simulink model "asbCubeSat"  (R2025b)
settings: Solver=VariableStepAuto  StartTime=0.0  StopTime=10800  FixedStep=CubeSatTimeStep  MaxStep=10  RelTol=1e-7  AbsTol=1e-7  EnableMultiTasking=on
libraries: simulink x12, aerolibutil x5, asbCubeSatEnvironmentLib x1, SignalEditorBlockLib x1, sharedutil x1, asbCubeSatActuatorsLib x1, asbCubeSatSensorsLib x1, asbCubeSatDynamicsLib x1, asbCubeSatFSWLib x1
settings Model: RequirementInfo={} %GIDa_aedc6be2_fb6a_446c_8c25_10b8bc9db182  DataDictionary=asbCubeSatModelData.sldd  SnapshotInterval=1  ExtModeAutoUpdateStatusClock=off  Creator=The MathWorks, Inc.  LastModifiedBy=The MathWorks, Inc.
settings SolverCC: AlgebraicLoopSolver=TrustRegion  MaxZcPerStep=1.0
settings DataIOCC: LimitDataPoints=on  SaveFormat=Array  SaveOutput=off  DSMLogging=off  SaveTime=off  ReturnWorkspaceOutputs=off
settings OptimizationCC: DefaultParameterBehavior=Inlined  OptimizeBlockIOStorage=off  BufferReuse=off  GlobalBufferReuse=off  ExpressionFolding=off  ExpressionDepthLimit=2147483647.0  LocalBlockOutputs=off  InitFltsAndDblsToZero=on  LifeSpan=inf  OptimizeDataStoreBuffers=off  BusAssignmentInplaceUpdate=off
settings DebuggingCC: SignalResolutionControl=TryResolveAllWithWarning  MultiTaskDSMMsg=warning  MultiTaskCondExecSysMsg=none  UnconnectedInputMsg=warning  UnconnectedOutputMsg=warning  UnconnectedLineMsg=warning  AssertControl=DisableAll  StateNameClashWarn=warning  PregeneratedLibrarySubsystemCodeDiagnostic=none  SFUnexpectedBacktrackingDiag=warning  SFNoUnconditionalDefaultTransitionDiag=warning  SFExecutionAtInitializationDiag=none  ArithmeticOperatorsInVariantConditions=warning
settings HardwareCC: ProdBitPerPointer=32.0  ProdBitPerSizeT=32.0  ProdBitPerPtrDiffT=32.0  ProdLargestAtomicFloat=None  ProdIntDivRoundTo=Undefined  ProdEndianess=Unspecified  ProdWordSize=32.0  ProdHWDeviceType=32-bit Generic
settings ModelReferenceCC: UpdateModelReferenceTargets=IfOutOfDate  EnableRefExpFcnMdlSchedulingChecks=on  ModelReferenceMinAlgLoopOccurrences=on  PropagateSignalLabelsOutOfModel=off
settings SFSimCC: SimUseLocalCustomCode=off
settings RTWCC: RTWUseLocalCustomCode=off  GPUComputeCapability=3.5  DLArmComputeVersion=19.05
settings CodeAppCC: StateflowObjectComments=on
settings GRTTargetCC: TargetFcnLib=ansi_tfl_tmw.mat  TargetLangStandard=C89/C90 (ANSI)  CombineOutputUpdateFcns=off  GRTInterface=on
settings ConfigComp: CovMetricSettings=dw  CovSaveCumulativeToWorkspaceVar=on  CovSaveSingleToWorkspaceVar=on  CovExternalEMLEnable=off

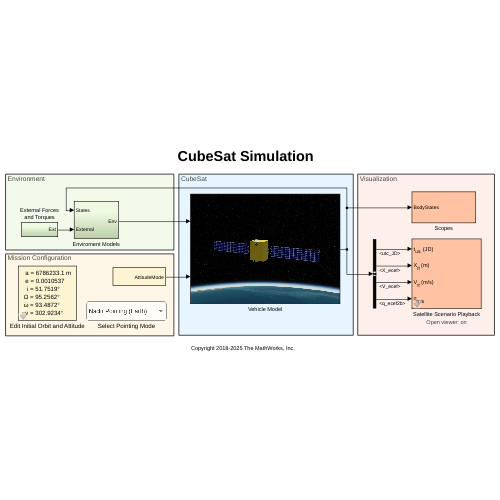
[thumbnail: Simulink's stored preview of the top-level diagram]
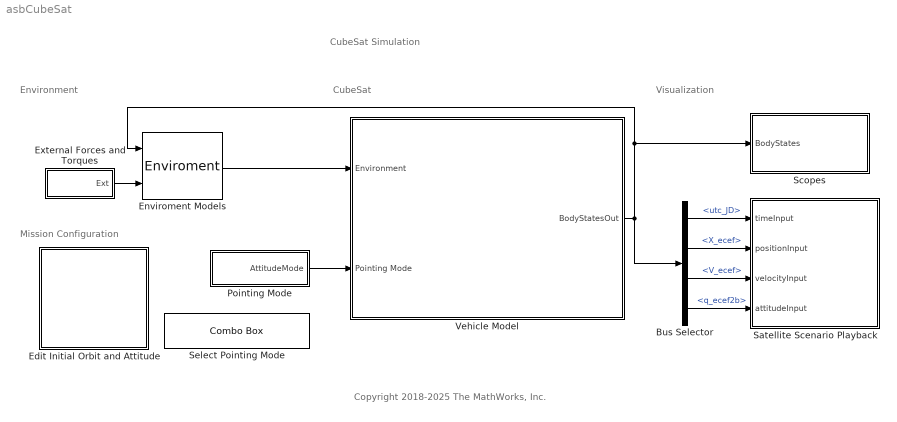
== system asbCubeSat ==
  note: Visualization
  note: CubeSat
  note: Environment
  note: Copyright 2018-2025 The MathWorks, Inc.
  note: CubeSat Simulation
  note: Mission Configuration
  Bus Selector : BusSelector  OutputSignals=utc_JD,X_ecef,V_ecef,q_ecef2b
  Edit Initial Orbit and Attitude : Subsystem  mask(CubeSat Initial Conditions){sim_t0=2458488, epoch=2451545, method=Keplerian Orbital Elements, a=6786233.13, ecc=0.0010537, incl=51.7519, omega=95.2562, argp=93.4872, nu=302.9234, truelon=0, arglat=0, lonper=0, r_eci=[-2981784.257 5207055.9381 3161595.3068], v_eci=[-3384.4834 -4887.7595 4843.4609], r_ecef=[-5762650.9114 -1682704.282 3156028.2879], v_ecef=[3832.57 -4024.9014 4837.4311], lla=[27.88080034 -163.722102 408851.6223], v_ned=[5468.7396 4937.8129 -7.4627367], euler=[33.9 -5.91 9.88], pqr=[0 0 0]}
      mask prompts: sim_t0 "spacecraft:cubesat:StartDate"; epoch "spacecraft:cubesat:ECIEpoch"; method "spacecraft:cubesat:InputMethod"; a "spacecraft:cubesat:SemiMajorAxis"; ecc "spacecraft:cubesat:Eccentricity"; incl "spacecraft:cubesat:Inclination"; omega "spacecraft:cubesat:RAAN"; argp "spacecraft:cubesat:ArgP"; nu "spacecraft:cubesat:TrueAnomaly"; truelon "spacecraft:cubesat:TrueLon"; arglat "spacecraft:cubesat:ArgLat"; lonper "spacecraft:cubesat:LonPer"; r_eci "spacecraft:cubesat:ECIPos"; v_eci "spacecraft:cubesat:ECIVel"; r_ecef "spacecraft:cubesat:ECEFPos"; v_ecef "spacecraft:cubesat:ECEFVel"; lla "spacecraft:cubesat:LLA"; v_ned "spacecraft:cubesat:NEDVel"; euler "spacecraft:cubesat:Euler"; pqr "spacecraft:cubesat:BodyAngRates"
      mask help: spacecraft:cubesat:InitCondBlockDesc
      mask init:
      | initCond = cubeSatCallback(gcb, 'computeIC', method, sim_t0, epoch, a, ecc, incl,...
      |     omega, argp, nu, truelon, arglat, lonper, r_eci, v_eci, r_ecef, v_ecef, lla,...
      |     v_ned, euler, pqr);
      mask TypeOptions method: spacecraft:cubesat:InputKeplerian | spacecraft:cubesat:InputECI | spacecraft:cubesat:InputECEF | spacecraft:cubesat:InputLLANED
      mask Callback method: cubeSatCallback(gcb, 'handleMethod');
      mask Callback ecc: cubeSatCallback(gcb, 'handleCircularOrbit');
      mask Callback incl: cubeSatCallback(gcb, 'handleCircularOrbit');
      mask DialogControl sim_t0 Prompt: Start date [Julian date]:
      mask DialogControl sim_t0 Tooltip: spacecraft:spacecraft:StartDateTT
      mask DialogControl icTab Prompt: spacecraft:cubesat:InitCond
      mask DialogControl epoch Prompt: Epoch of ECI frame [Julian date]:
      mask DialogControl epoch Tooltip: spacecraft:cubesat:ECIEpochTT
      mask DialogControl Container9 Prompt: spacecraft:cubesat:InitCondOrbit
      mask DialogControl method Prompt: Input method:
      mask DialogControl method Tooltip: spacecraft:cubesat:InputMethodTT
      mask DialogControl a Prompt: Semi-major axis [m]:
      mask DialogControl a Tooltip: spacecraft:cubesat:SemiMajorAxisTT
      mask DialogControl ecc Prompt: Eccentricity:
      mask DialogControl ecc Tooltip: spacecraft:cubesat:EccentricityTT
      mask DialogControl incl Prompt: Inclination [deg]:
      mask DialogControl incl Tooltip: spacecraft:cubesat:InclinationTT
      mask DialogControl omega Prompt: Right ascension of the ascending node [deg]:
      mask DialogControl omega Tooltip: spacecraft:cubesat:RAANTT
      mask DialogControl argp Prompt: Argument of periapsis [deg]:
      mask DialogControl argp Tooltip: spacecraft:cubesat:ArgPTT
      mask DialogControl nu Prompt: True anomaly [deg]:
      mask DialogControl nu Tooltip: spacecraft:cubesat:TrueAnomalyTT
      mask DialogControl truelon Prompt: True longitude [deg] (circular equatorial):
      mask DialogControl truelon Tooltip: spacecraft:cubesat:TrueLonTT
      mask DialogControl arglat Prompt: Argument of latitude [deg] (circular inclined):
      mask DialogControl arglat Tooltip: spacecraft:cubesat:ArgLatTT
      mask DialogControl lonper Prompt: Longitude of periapsis [deg] (elliptical equatorial):
      mask DialogControl lonper Tooltip: spacecraft:cubesat:LonPerTT
      mask DialogControl r_eci Prompt: ECI position vector [m]:
      mask DialogControl r_eci Tooltip: spacecraft:cubesat:ECIPosTT
      mask DialogControl v_eci Prompt: ECI velocity vector [m/s]:
      mask DialogControl v_eci Tooltip: spacecraft:cubesat:ECIVelTT
      mask DialogControl r_ecef Prompt: ECEF position vector [m]:
      mask DialogControl r_ecef Tooltip: spacecraft:cubesat:ECEFPosTT
      mask DialogControl v_ecef Prompt: ECEF velocity vector [m/s]:
      mask DialogControl v_ecef Tooltip: spacecraft:cubesat:ECEFVelTT
      mask DialogControl lla Prompt: Geodetic latitude, longitude, altitude [deg, deg, m]:
      mask DialogControl lla Tooltip: spacecraft:cubesat:LLATT
      mask DialogControl v_ned Prompt: NED velocity vector [m/s]:
      mask DialogControl v_ned Tooltip: spacecraft:cubesat:NEDVelTT
      mask DialogControl Container11 Prompt: spacecraft:cubesat:InitCondAttitude
      mask DialogControl euler Prompt: Initial Euler angles (roll, pitch, yaw) [deg]:
      mask DialogControl euler Tooltip: spacecraft:cubesat:EulerTT
      mask DialogControl pqr Prompt: Initial body angular rates [deg/s]:
      mask DialogControl pqr Tooltip: spacecraft:cubesat:BodyAngRatesTT
      mask Display:
      | text(.1, .9, [' a = ' sprintf('%.1f', str2double(get_param(gcb, 'a'))) ' m'],'horizontalAlignment','left','texmode','on');
      | text(.1, .75, [' e = ' get_param(gcb, 'ecc')],'horizontalAlignment','left','texmode', 'on')
      | text(.1, .6, ['  i = ' get_param(gcb, 'incl') '\circ'],'horizontalAlignment','left','texmode', 'on')
      | text(.1, .45, ['\Omega = ' get_param(gcb, 'omega') '\circ'],'horizontalAlignment','left','texmode', 'on')
      | text(.1, .3, ['\omega = ' get_param(gcb, 'argp') '\circ'],'horizontalAlignment','left','texmode', 'on')
      | text(.1, .15, [' \nu = ' get_param(gcb, 'nu') '\circ'],'horizontalAlignment','left','texmode', 'on')
  Enviroment Models : asbCubeSatEnvironmentLib/Enviroment  SystemSampleTime=-1  VariantActivationTime=update diagram  EmptyChoice=off  PassThrough=off  PassThroughVariantControl=(default)  EmptyChoiceVariantControl=(default)  AllowFlexibleInterface=on  Latency=0  AutoFrameSizeCalculation=off
  "External Forces and Torques " : Subsystem
  Pointing Mode : Subsystem
  Satellite Scenario Playback : Subsystem  StopFcn=|  mask{openViewer=on, stateFrame=ECEF (Fixed-frame), useVelocity=on, useAttitude=on, attitudeFrame=ECEF (Fixed-frame), satName=Satellite, showTriad=on, show3dModel=on, showFOV=on, fovHalfAngle=30, scenarioStep=60}
      | exSatScenBlk = gcb;
      | exSatScenMdl = bdroot(exSatScenBlk);
      | 
      | % If workspace blocks are stored in single output variable, need to access from there
      | if get_param(exSatScenMdl, "ReturnWorkspaceOutputs") == "on"
      |     exSatScenOutVar = get_param(exSatScenMdl, "ReturnWorkspaceOutputsName");
      |     if exist(exSatScenOutVar)
      |         exSatScenTimeData = eval(exSatScenOutVar).exSatScenTimeData;
      |         exSatScenPositionData = eval(exSatScenOutVar).exSatScenPositionData;
      |         exSatScenVelocityData = eval(exSatScenOutVar).exSatScenVelocityData;
      |         exSatScenAttitudeData = eval(exSatScenOutVar).exSatScenAttitudeData;
      |     end
      | end
      | 
      | % If variables exist, create scenario (variables are not created if called with sim command)
      | if exist("exSatScenTimeData") && exist("exSatScenPositionData") && exist("exSatScenVelocityData") && exist("exSatScenAttitudeData") 
      |     % Create satellite scenario from variables accessed above or directly from workspace
      |     exSatScenario = Aero.spacecraft.analysis.createSatelliteScenarioFromSim(exSatScenBlk, ...
      |         exSatScenTimeData, exSatScenPositionData, exSatScenVelocityData, exSatScenAttitudeData);
      | end
      | 
      | clear exSatScenBlk exSatScenMdl exSatScenOutVar exSatScenTimeData exSatScenPositionData exSatScenVelocityData exSatScenAttitudeData
      mask prompts: openViewer "Enable Satellite Scenario Viewer playback animation"; stateFrame "State coordinate frame:"; useVelocity "Add velocity port"; useAttitude "Add attitude port"; attitudeFrame "Attitude coordinate frame (Frame to Body):"; satName "Satellite or constellation label:"; showTriad "Show coordinate axis triad (Body frame)"; show3dModel "Show 3D satellite model"; showFOV "Add sensor field-of-view (FOV)"; fovHalfAngle "FOV half angle (deg):"; scenarioStep "Satellite scenario sample time (s):"
      mask init:
      | ports = Aero.spacecraft.analysis.satelliteScenarioPlaybackMaskCallback(gcb, "init");
      settings: AttributesFormatString=Open viewer: %<openViewer>
      mask Callback openViewer: Aero.spacecraft.analysis.satelliteScenarioPlaybackMaskCallback(gcb, "viewer");
      mask TypeOptions stateFrame: Inertial (ICRF) | ECEF (Fixed-frame) | Geographic
      mask Callback useAttitude: Aero.spacecraft.analysis.satelliteScenarioPlaybackMaskCallback(gcb, "attitude");
      mask TypeOptions attitudeFrame: Inertial (ICRF) | ECEF (Fixed-frame) | NED
      mask Callback showFOV: Aero.spacecraft.analysis.satelliteScenarioPlaybackMaskCallback(gcb, "fov");
      mask DialogControl DescGroupVar Prompt: Satellite Scenario Viewer Playback Animation
      mask DialogControl DescTextVar Prompt: <html><p>Create a satelliteScenario object and open Satellite Scenario Viewer using the trajectories provided as inputs to the block.</p><p>If playback animation is enabled, Satellite Scenario Viewer is opened after the model simulation stops. To start the simulation, click the Run button. Using the <tt>sim</tt> function does not open the viewer.</p><p>To add additional satellites, ground stations, or platforms to the scenario, and perform mission analysis such as line-of-sight access and eclipse analysis, use the base workspace variable <tt>exSatScenario</tt>.</p></html>
      mask DialogControl Container3 Prompt: Parameters
      mask DialogControl Container4 Prompt: Trajectory
      mask DialogControl ParameterGroupVar Prompt: Playback
      mask DialogControl SatelliteScenarioPlaybackTag Prompt: SatelliteScenarioPlaybackTag
      mask Display:
      | port_label(ports(1).type,ports(1).port,ports(1).txt,'texmode','on');
      | port_label(ports(2).type,ports(2).port,ports(2).txt,'texmode','on');
      | port_label(ports(3).type,ports(3).port,ports(3).txt,'texmode','on');
      | port_label(ports(4).type,ports(4).port,ports(4).txt,'texmode','on');
  Scopes : Subsystem  VariantControl=visOff
  Select Pointing Mode : ComboBox  LabelPosition=Hide  SelectedLabel=Nadir Pointing (Earth)
  Vehicle Model : Subsystem
      mask Display: image('CubeSatVehicle.PNG');
  wires:
  Enviroment Models/1 -> Vehicle Model/1(Environment)
  "External Forces and Torques "/1(Ext) -> Enviroment Models/2
  Vehicle Model/1(BodyStatesOut) -> Bus Selector/1, Scopes/1(BodyStates), Enviroment Models/1
  Pointing Mode/1(AttitudeMode) -> Vehicle Model/2(Pointing Mode)
  Bus Selector/1 -> Satellite Scenario Playback/1(timeInput)  "<utc_JD>"
  Bus Selector/2 -> Satellite Scenario Playback/2(positionInput)  "<X_ecef>"
  Bus Selector/3 -> Satellite Scenario Playback/3(velocityInput)  "<V_ecef>"
  Bus Selector/4 -> Satellite Scenario Playback/4(attitudeInput)  "<q_ecef2b>"

== system asbCubeSat/Edit Initial Orbit and Attitude ==

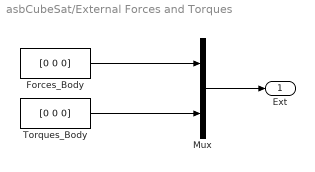
== system asbCubeSat/External Forces and Torques  ==
  Forces_Body : Constant  Value=[0 0 0]
  Mux : Mux  RequirementInfo={} %GIDa_ef4ca723_4eef_40f8_bb1e_99de60d2b248  Inputs=2
  Torques_Body : Constant  Value=[0 0 0]
  Ext : Outport  RequirementInfo={} %GIDa_0f078eca_6127_499d_b81c_658503a40261  VectorParamsAs1DForOutWhenUnconnected=off
  wires:
  Forces_Body/1 -> Mux/1
  Torques_Body/1 -> Mux/2
  Mux/1 -> Ext/1

== system asbCubeSat/Pointing Mode ==
  note: Modes:
      | 0 = Off
      | 1 = Earth (Nadir)
      | 2 = Sun
  Mode : Constant  SampleTime=-1
  Multiport Switch : MultiPortSwitch  DataPortOrder=Specify indices  DataPortIndices={3, [0,1,2]}  DiagnosticForDefault=None  SaturateOnIntegerOverflow=off  InputSameDT=off
  Signal Editor : SignalEditorBlockLib/Signal Editor  FileName=SignalEditorPointing.mat  ActiveScenario=PointingScenario  ActiveSignal=PointingMode  IsBus=off  OutputBusObjectStr=Bus: BusObject  SampleTime=0  Interpolate=off  ZeroCross=off  OutputAfterFinalValue=Setting to zero  Unit=inherit  PreserveSignalName=on  ApplySigPropsToAllScenarios=on  ApplySigPropsToAllSignals=off  SignalPropertySource=Dialog parameters
  AttitudeMode : Outport  VectorParamsAs1DForOutWhenUnconnected=off
  wires:
  Signal Editor/1 -> Multiport Switch/2
  Mode/1 -> Multiport Switch/1, Multiport Switch/3
  Multiport Switch/1 -> AttitudeMode/1

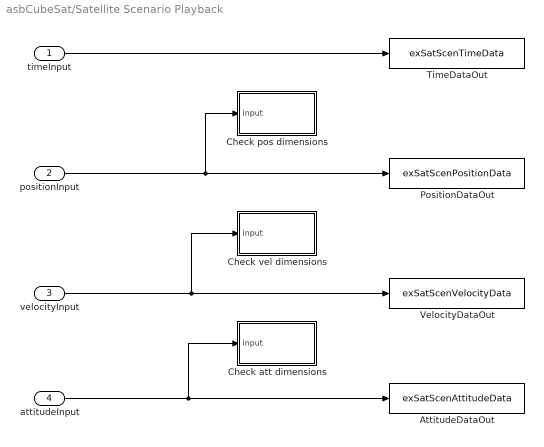
== system asbCubeSat/Satellite Scenario Playback ==
  timeInput : Inport  PortDimensions=1
  positionInput : Inport  Port=2  Unit=m
  velocityInput : Inport  Port=3  Unit=m/s
  attitudeInput : Inport  Port=4
  AttitudeDataOut : ToWorkspace  VariableName=exSatScenAttitudeData  SampleTime=-1
  Check att dimensions : Subsystem  mask{N=4, AssertionFailFcn=error("Attitude input must be be a vector with 4 elements or a 2-D array of size [m x 4].")}
      mask prompts: N "State dimension (N):"; AssertionFailFcn "Simulink:blkprm_prompts:AssertionCallback"
      mask TypeOptions AssertionFailFcn: Assertion/AssertionFailFcn | Second check/Assertion/AssertionFailFcn
      mask DialogControl DescGroupVar Prompt: Assert expected dimensions
      mask DialogControl DescTextVar Prompt: Assert that input signal is size N or size M x N where M is the number of satellites. N is 3 for position and velocity, and 4 for attitude (quaternions).
      mask DialogControl AssertionFailFcn Prompt: Simulation callback when assertion fails:
  Check pos dimensions : Subsystem  mask{N=3, AssertionFailFcn=error("Position input must be be a vector with 3 elements or a 2-D array of size [m x 3].")}
      mask prompts: N "State dimension (N):"; AssertionFailFcn "Simulink:blkprm_prompts:AssertionCallback"
      mask TypeOptions AssertionFailFcn: Assertion/AssertionFailFcn | Second check/Assertion/AssertionFailFcn
      mask DialogControl DescGroupVar Prompt: Assert expected dimensions
      mask DialogControl DescTextVar Prompt: Assert that input signal is size N or size M x N where M is the number of satellites. N is 3 for position and velocity, and 4 for attitude (quaternions).
      mask DialogControl AssertionFailFcn Prompt: Simulation callback when assertion fails:
  Check vel dimensions : Subsystem  mask{N=3, AssertionFailFcn=error("Velocity input must be be a vector with 3 elements or a 2-D array of size [m x 3].")}
      mask prompts: N "State dimension (N):"; AssertionFailFcn "Simulink:blkprm_prompts:AssertionCallback"
      mask TypeOptions AssertionFailFcn: Assertion/AssertionFailFcn | Second check/Assertion/AssertionFailFcn
      mask DialogControl DescGroupVar Prompt: Assert expected dimensions
      mask DialogControl DescTextVar Prompt: Assert that input signal is size N or size M x N where M is the number of satellites. N is 3 for position and velocity, and 4 for attitude (quaternions).
      mask DialogControl AssertionFailFcn Prompt: Simulation callback when assertion fails:
  PositionDataOut : ToWorkspace  VariableName=exSatScenPositionData  SampleTime=-1
  TimeDataOut : ToWorkspace  VariableName=exSatScenTimeData  SampleTime=-1
  VelocityDataOut : ToWorkspace  VariableName=exSatScenVelocityData  SampleTime=-1
  wires:
  timeInput/1 -> TimeDataOut/1
  attitudeInput/1 -> AttitudeDataOut/1, Check att dimensions/1(input)
  velocityInput/1 -> VelocityDataOut/1, Check vel dimensions/1(input)
  positionInput/1 -> Check pos dimensions/1(input), PositionDataOut/1

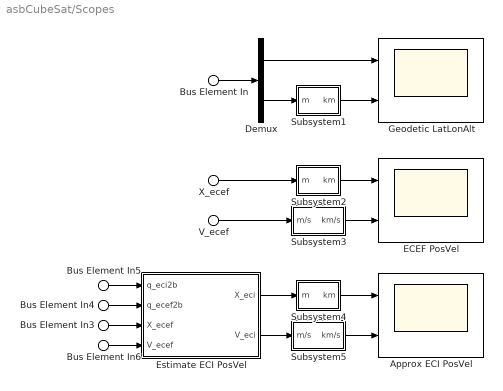
== system asbCubeSat/Scopes ==
  Bus Element In : Inport  PortName=BodyStates  Element=LatLonAlt
  X_ecef : Inport  PortName=BodyStates  Element=X_ecef
  Bus Element In3 : Inport  PortName=BodyStates  Element=X_ecef
  V_ecef : Inport  PortName=BodyStates  Element=V_ecef
  Bus Element In6 : Inport  PortName=BodyStates  Element=V_ecef
  Bus Element In4 : Inport  PortName=BodyStates  Element=q_ecef2b
  Bus Element In5 : Inport  PortName=BodyStates  Element=q_eci2b
  Approx ECI PosVel : Scope  NumInputPorts=2
      settings: Title=Earth-centered Inertial Position  ActiveDisplayYMinimum=-8479.67563  ActiveDisplayYMaximum=8481.52428  YLabel=X_{ECI} (km)
  Demux : Demux  Outputs=[2 1]
  ECEF PosVel : Scope  NumInputPorts=2
      settings: Title=Earth-centered Earth-fixed Position  ActiveDisplayYMinimum=-8477.4718  ActiveDisplayYMaximum=8446.48345  YLabel=X_{ECEF} (km)  DataLoggingVariableName=ScopeData2
  Estimate ECI PosVel : Subsystem
  Geodetic LatLonAlt : Scope  NumInputPorts=2
      settings: Title=Geodetic Latitude and Longitude  ActiveDisplayYMinimum=-224.99763  ActiveDisplayYMaximum=224.99581  YLabel=\mu \iota (deg)
  Subsystem1 : Subsystem
  Subsystem2 : Subsystem
  Subsystem3 : Subsystem
  Subsystem4 : Subsystem
  Subsystem5 : Subsystem
  wires:
  Bus Element In/1 -> Demux/1
  Demux/1 -> Geodetic LatLonAlt/1
  Demux/2 -> Subsystem1/1(m)
  X_ecef/1 -> Subsystem2/1(m)
  V_ecef/1 -> Subsystem3/1(m/s)
  Estimate ECI PosVel/1(X_eci) -> Subsystem4/1(m)
  Estimate ECI PosVel/2(V_eci) -> Subsystem5/1(m/s)
  Bus Element In5/1 -> Estimate ECI PosVel/1(q_eci2b)
  Bus Element In4/1 -> Estimate ECI PosVel/2(q_ecef2b)
  Bus Element In3/1 -> Estimate ECI PosVel/3(X_ecef)
  Bus Element In6/1 -> Estimate ECI PosVel/4(V_ecef)
  Subsystem1/1(km) -> Geodetic LatLonAlt/2
  Subsystem2/1(km) -> ECEF PosVel/1
  Subsystem3/1(km/s) -> ECEF PosVel/2
  Subsystem4/1(km) -> Approx ECI PosVel/1
  Subsystem5/1(km/s) -> Approx ECI PosVel/2

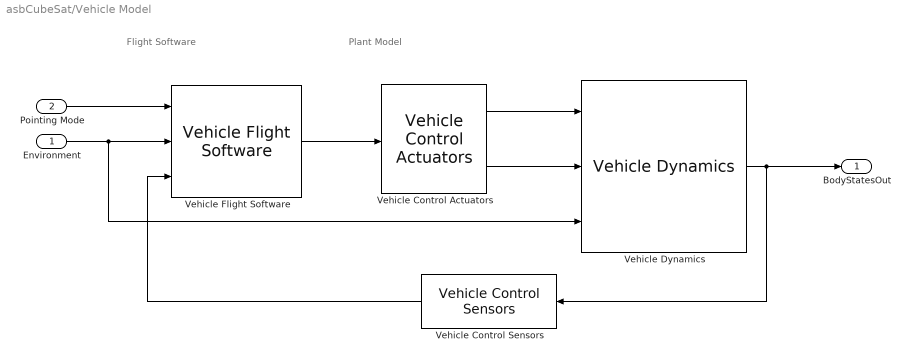
== system asbCubeSat/Vehicle Model ==
  note: Flight Software
  note: Plant Model
  Environment : Inport
  Pointing Mode : Inport  Port=2
  Vehicle Control Actuators : asbCubeSatActuatorsLib/Vehicle Control Actuators  SystemSampleTime=-1  VariantActivationTime=update diagram  EmptyChoice=off  PassThrough=off  PassThroughVariantControl=(default)  EmptyChoiceVariantControl=(default)  AllowFlexibleInterface=on  Latency=0  AutoFrameSizeCalculation=off
  Vehicle Control Sensors : asbCubeSatSensorsLib/Vehicle Control Sensors  SystemSampleTime=-1  VariantActivationTime=update diagram  EmptyChoice=off  PassThrough=off  PassThroughVariantControl=(default)  EmptyChoiceVariantControl=(default)  AllowFlexibleInterface=on  Latency=0  AutoFrameSizeCalculation=off
  Vehicle Dynamics : asbCubeSatDynamicsLib/Vehicle Dynamics  SystemSampleTime=-1  VariantActivationTime=update diagram  EmptyChoice=off  PassThrough=off  PassThroughVariantControl=(default)  EmptyChoiceVariantControl=(default)  AllowFlexibleInterface=on  Latency=0  AutoFrameSizeCalculation=off
  Vehicle Flight Software : asbCubeSatFSWLib/Vehicle Flight Software  SystemSampleTime=-1  VariantActivationTime=update diagram  EmptyChoice=off  PassThrough=off  PassThroughVariantControl=(default)  EmptyChoiceVariantControl=(default)  AllowFlexibleInterface=on  Latency=0  AutoFrameSizeCalculation=off
  BodyStatesOut : Outport  OutDataTypeStr=Bus: StatesOutBus  VectorParamsAs1DForOutWhenUnconnected=off
  wires:
  Vehicle Dynamics/1 -> Vehicle Control Sensors/1, BodyStatesOut/1
  Pointing Mode/1 -> Vehicle Flight Software/1
  Vehicle Control Sensors/1 -> Vehicle Flight Software/3
  Vehicle Control Actuators/1 -> Vehicle Dynamics/1
  Vehicle Control Actuators/2 -> Vehicle Dynamics/2
  Vehicle Flight Software/1 -> Vehicle Control Actuators/1
  Environment/1 -> Vehicle Dynamics/3, Vehicle Flight Software/2

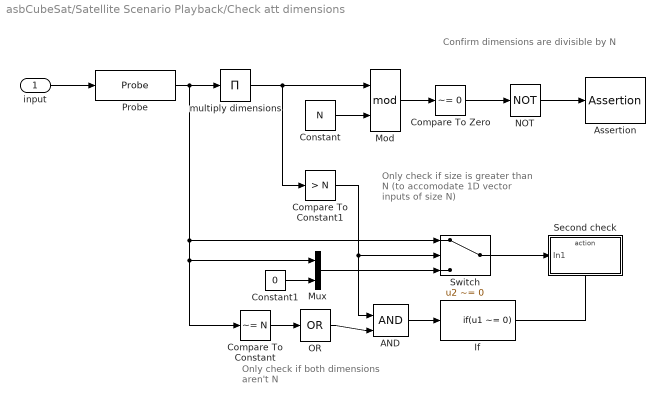
== system asbCubeSat/Satellite Scenario Playback/Check att dimensions ==
  note: Confirm dimensions are divisible by N
  note: Only check if size is greater than N (to accomodate 1D vector inputs of size N)
  note: Only check if both dimensions aren't N
  input : Inport
  AND : Logic  IconShape=distinctive  AllPortsSameDT=off  OutDataTypeStr=boolean
  Assertion : Assertion  AssertionFailFcn="error(\"Attitude input must be be a vector with 4 elements or a 2-D array of size [m x 4].\")"
  Compare To Constant : simulink/Logic and Bit Operations/Compare To Constant  relop=~=  const=N  OutDataTypeStr=boolean  ZeroCross=off
  Compare To Constant1 : simulink/Logic and Bit Operations/Compare To Constant  relop=>  const=N  OutDataTypeStr=boolean  ZeroCross=off
  Compare To Zero : simulink/Logic and Bit Operations/Compare To Zero  relop=~=  OutDataTypeStr=boolean  ZeroCross=off
  Constant : Constant  Value=N  OutDataTypeStr=uint8
  Constant1 : Constant  Value=0  OutDataTypeStr=uint8
  If : If  IfExpression=u1 ~= 0  ShowElse=off  ZeroCross=off
  Mod : Math  Operator=mod
  Mux : Mux  Inputs=2
  NOT : Logic  Operator=NOT  IconShape=distinctive  AllPortsSameDT=off  OutDataTypeStr=boolean
  OR : Logic  Operator=OR  Inputs=1  IconShape=distinctive  AllPortsSameDT=off  OutDataTypeStr=boolean
  Probe : Probe  ProbeWidth=off  ProbeSampleTime=off  ProbeComplexSignal=off  ProbeSignalDimensions=on  ProbeDimensionsDataType=uint8
  Second check : Subsystem  TreatAsAtomicUnit=on
  Switch : Switch  Criteria=u2 ~= 0  SaturateOnIntegerOverflow=off  InputSameDT=off
  multiply dimensions : Product  Inputs=*  OutDataTypeStr=uint8
  wires:
  Switch/1 -> Second check/1(In1)
  Mux/1 -> Switch/3
  Constant1/1 -> Mux/2
  AND/1 -> If/1
  Compare To Constant1/1 -> AND/1, Switch/2
  If/1 -> Second check/Action
  OR/1 -> AND/2
  Compare To Constant/1 -> OR/1
  Probe/1 -> multiply dimensions/1, Switch/1, Compare To Constant/1, Mux/1
  multiply dimensions/1 -> Mod/1, Compare To Constant1/1
  NOT/1 -> Assertion/1
  Mod/1 -> Compare To Zero/1
  Compare To Zero/1 -> NOT/1
  Constant/1 -> Mod/2
  input/1 -> Probe/1

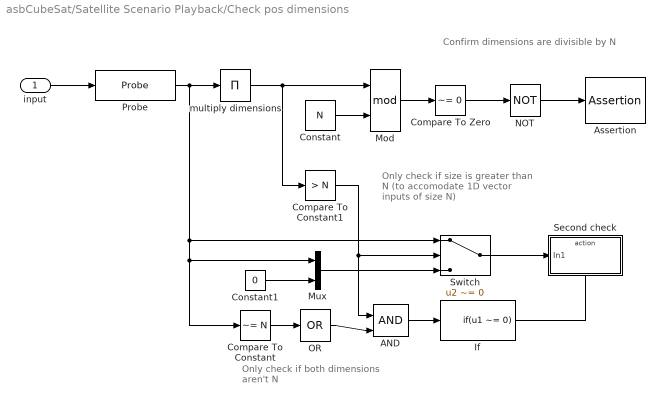
== system asbCubeSat/Satellite Scenario Playback/Check pos dimensions ==
  note: Confirm dimensions are divisible by N
  note: Only check if size is greater than N (to accomodate 1D vector inputs of size N)
  note: Only check if both dimensions aren't N
  input : Inport
  AND : Logic  IconShape=distinctive  AllPortsSameDT=off  OutDataTypeStr=boolean
  Assertion : Assertion  AssertionFailFcn="error(\"Position input must be be a vector with 3 elements or a 2-D array of size [m x 3].\")"
  Compare To Constant : simulink/Logic and Bit Operations/Compare To Constant  relop=~=  const=N  OutDataTypeStr=boolean  ZeroCross=off
  Compare To Constant1 : simulink/Logic and Bit Operations/Compare To Constant  relop=>  const=N  OutDataTypeStr=boolean  ZeroCross=off
  Compare To Zero : simulink/Logic and Bit Operations/Compare To Zero  relop=~=  OutDataTypeStr=boolean  ZeroCross=off
  Constant : Constant  Value=N  OutDataTypeStr=uint8
  Constant1 : Constant  Value=0  OutDataTypeStr=uint8
  If : If  IfExpression=u1 ~= 0  ShowElse=off  ZeroCross=off
  Mod : Math  Operator=mod
  Mux : Mux  Inputs=2
  NOT : Logic  Operator=NOT  IconShape=distinctive  AllPortsSameDT=off  OutDataTypeStr=boolean
  OR : Logic  Operator=OR  Inputs=1  IconShape=distinctive  AllPortsSameDT=off  OutDataTypeStr=boolean
  Probe : Probe  ProbeWidth=off  ProbeSampleTime=off  ProbeComplexSignal=off  ProbeSignalDimensions=on  ProbeDimensionsDataType=uint8
  Second check : Subsystem  TreatAsAtomicUnit=on
  Switch : Switch  Criteria=u2 ~= 0  SaturateOnIntegerOverflow=off  InputSameDT=off
  multiply dimensions : Product  Inputs=*  OutDataTypeStr=uint8
  wires:
  Switch/1 -> Second check/1(In1)
  Mux/1 -> Switch/3
  Constant1/1 -> Mux/2
  AND/1 -> If/1
  Compare To Constant1/1 -> AND/1, Switch/2
  If/1 -> Second check/Action
  OR/1 -> AND/2
  Compare To Constant/1 -> OR/1
  Probe/1 -> multiply dimensions/1, Switch/1, Compare To Constant/1, Mux/1
  multiply dimensions/1 -> Mod/1, Compare To Constant1/1
  NOT/1 -> Assertion/1
  Mod/1 -> Compare To Zero/1
  Compare To Zero/1 -> NOT/1
  Constant/1 -> Mod/2
  input/1 -> Probe/1

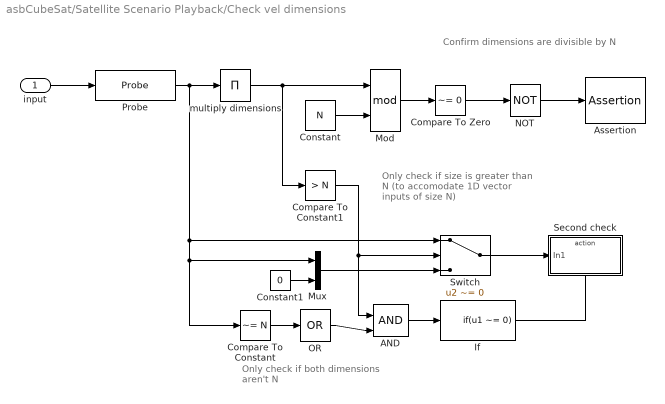
== system asbCubeSat/Satellite Scenario Playback/Check vel dimensions ==
  note: Only check if both dimensions aren't N
  note: Only check if size is greater than N (to accomodate 1D vector inputs of size N)
  note: Confirm dimensions are divisible by N
  input : Inport
  AND : Logic  IconShape=distinctive  AllPortsSameDT=off  OutDataTypeStr=boolean
  Assertion : Assertion  AssertionFailFcn="error(\"Velocity input must be be a vector with 3 elements or a 2-D array of size [m x 3].\")"
  Compare To Constant : simulink/Logic and Bit Operations/Compare To Constant  relop=~=  const=N  OutDataTypeStr=boolean  ZeroCross=off
  Compare To Constant1 : simulink/Logic and Bit Operations/Compare To Constant  relop=>  const=N  OutDataTypeStr=boolean  ZeroCross=off
  Compare To Zero : simulink/Logic and Bit Operations/Compare To Zero  relop=~=  OutDataTypeStr=boolean  ZeroCross=off
  Constant : Constant  Value=N  OutDataTypeStr=uint8
  Constant1 : Constant  Value=0  OutDataTypeStr=uint8
  If : If  IfExpression=u1 ~= 0  ShowElse=off  ZeroCross=off
  Mod : Math  Operator=mod
  Mux : Mux  Inputs=2
  NOT : Logic  Operator=NOT  IconShape=distinctive  AllPortsSameDT=off  OutDataTypeStr=boolean
  OR : Logic  Operator=OR  Inputs=1  IconShape=distinctive  AllPortsSameDT=off  OutDataTypeStr=boolean
  Probe : Probe  ProbeWidth=off  ProbeSampleTime=off  ProbeComplexSignal=off  ProbeSignalDimensions=on  ProbeDimensionsDataType=uint8
  Second check : Subsystem  TreatAsAtomicUnit=on
  Switch : Switch  Criteria=u2 ~= 0  SaturateOnIntegerOverflow=off  InputSameDT=off
  multiply dimensions : Product  Inputs=*  OutDataTypeStr=uint8
  wires:
  input/1 -> Probe/1
  Constant/1 -> Mod/2
  Compare To Zero/1 -> NOT/1
  Mod/1 -> Compare To Zero/1
  NOT/1 -> Assertion/1
  multiply dimensions/1 -> Compare To Constant1/1, Mod/1
  Probe/1 -> Mux/1, Compare To Constant/1, Switch/1, multiply dimensions/1
  Compare To Constant/1 -> OR/1
  OR/1 -> AND/2
  If/1 -> Second check/Action
  Compare To Constant1/1 -> Switch/2, AND/1
  AND/1 -> If/1
  Constant1/1 -> Mux/2
  Mux/1 -> Switch/3
  Switch/1 -> Second check/1(In1)

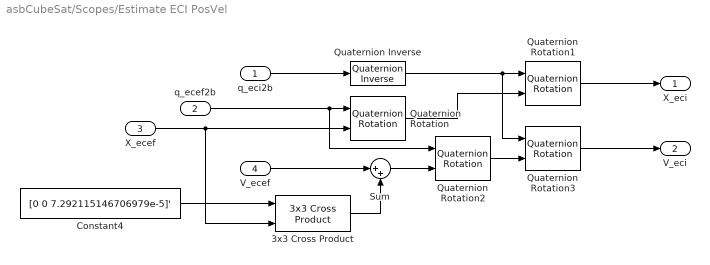
== system asbCubeSat/Scopes/Estimate ECI PosVel ==
  q_eci2b : Inport
  q_ecef2b : Inport  Port=2
  X_ecef : Inport  Port=3
  V_ecef : Inport  Port=4
  3x3 Cross Product : sharedutil/3x3 Cross Product  aMode=aMode
  Constant4 : Constant  Value=[0 0 7.292115146706979e-5]'
  Quaternion Inverse : aerolibutil/Quaternion Inverse
  Quaternion Rotation{,1..3} (4 alike) : aerolibutil/Quaternion Rotation
  Sum : Sum  Inputs=|++
  X_eci : Outport  VectorParamsAs1DForOutWhenUnconnected=off
  V_eci : Outport  Port=2  VectorParamsAs1DForOutWhenUnconnected=off
  wires:
  Sum/1 -> Quaternion Rotation2/2
  3x3 Cross Product/1 -> Sum/2
  V_ecef/1 -> Sum/1
  Quaternion Rotation/1 -> Quaternion Rotation1/2
  q_ecef2b/1 -> Quaternion Rotation/1, Quaternion Rotation2/1
  Quaternion Inverse/1 -> Quaternion Rotation3/1, Quaternion Rotation1/1
  Constant4/1 -> 3x3 Cross Product/1
  Quaternion Rotation2/1 -> Quaternion Rotation3/2
  q_eci2b/1 -> Quaternion Inverse/1
  Quaternion Rotation1/1 -> X_eci/1
  X_ecef/1 -> 3x3 Cross Product/2, Quaternion Rotation/2
  Quaternion Rotation3/1 -> V_eci/1

== system asbCubeSat/Scopes/Subsystem1 ==
  m : Inport  Unit=m
  Unit Conversion : UnitConversion
  km : Outport  Unit=km  VectorParamsAs1DForOutWhenUnconnected=off
  wires:
  m/1 -> Unit Conversion/1
  Unit Conversion/1 -> km/1

== system asbCubeSat/Scopes/Subsystem2 ==
  m : Inport  Unit=m
  Unit Conversion : UnitConversion
  km : Outport  Unit=km  VectorParamsAs1DForOutWhenUnconnected=off
  wires:
  Unit Conversion/1 -> km/1
  m/1 -> Unit Conversion/1

== system asbCubeSat/Scopes/Subsystem3 ==
  m/s : Inport  Unit=m/s
  Unit Conversion : UnitConversion
  km/s : Outport  Unit=km/s  VectorParamsAs1DForOutWhenUnconnected=off
  wires:
  m/s/1 -> Unit Conversion/1
  Unit Conversion/1 -> km/s/1

== system asbCubeSat/Scopes/Subsystem4 ==
  m : Inport  Unit=m
  Unit Conversion : UnitConversion
  km : Outport  Unit=km  VectorParamsAs1DForOutWhenUnconnected=off
  wires:
  Unit Conversion/1 -> km/1
  m/1 -> Unit Conversion/1

== system asbCubeSat/Scopes/Subsystem5 ==
  m/s : Inport  Unit=m/s
  Unit Conversion : UnitConversion
  km/s : Outport  Unit=km/s  VectorParamsAs1DForOutWhenUnconnected=off
  wires:
  m/s/1 -> Unit Conversion/1
  Unit Conversion/1 -> km/s/1

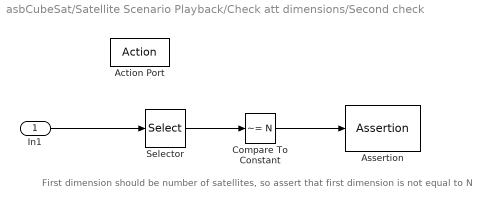
== system asbCubeSat/Satellite Scenario Playback/Check att dimensions/Second check ==
  note: First dimension should be number of satellites, so assert that first dimension is not equal to N
  In1 : Inport
  Action Port : ActionPort  ActionPortLabel=if(u1 ~= 0)
  Assertion : Assertion  AssertionFailFcn="error(\"Attitude input must be be a vector with 4 elements or a 2-D array of size [m x 4].\")"
  Compare To Constant : simulink/Logic and Bit Operations/Compare To Constant  relop=~=  const=N  OutDataTypeStr=boolean  ZeroCross=off
  Selector : Selector  InputPortWidth=2  IndexOptions=Index vector (dialog)  Indices=[1]  OutputSizes=1
  wires:
  Compare To Constant/1 -> Assertion/1
  In1/1 -> Selector/1
  Selector/1 -> Compare To Constant/1

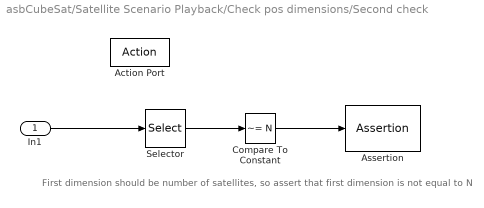
== system asbCubeSat/Satellite Scenario Playback/Check pos dimensions/Second check ==
  note: First dimension should be number of satellites, so assert that first dimension is not equal to N
  In1 : Inport
  Action Port : ActionPort  ActionPortLabel=if(u1 ~= 0)
  Assertion : Assertion  AssertionFailFcn="error(\"Position input must be be a vector with 3 elements or a 2-D array of size [m x 3].\")"
  Compare To Constant : simulink/Logic and Bit Operations/Compare To Constant  relop=~=  const=N  OutDataTypeStr=boolean  ZeroCross=off
  Selector : Selector  InputPortWidth=2  IndexOptions=Index vector (dialog)  Indices=[1]  OutputSizes=1
  wires:
  Compare To Constant/1 -> Assertion/1
  In1/1 -> Selector/1
  Selector/1 -> Compare To Constant/1

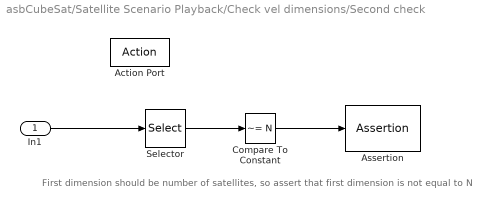
== system asbCubeSat/Satellite Scenario Playback/Check vel dimensions/Second check ==
  note: First dimension should be number of satellites, so assert that first dimension is not equal to N
  In1 : Inport
  Action Port : ActionPort  ActionPortLabel=if(u1 ~= 0)
  Assertion : Assertion  AssertionFailFcn="error(\"Velocity input must be be a vector with 3 elements or a 2-D array of size [m x 3].\")"
  Compare To Constant : simulink/Logic and Bit Operations/Compare To Constant  relop=~=  const=N  OutDataTypeStr=boolean  ZeroCross=off
  Selector : Selector  InputPortWidth=2  IndexOptions=Index vector (dialog)  Indices=[1]  OutputSizes=1
  wires:
  Selector/1 -> Compare To Constant/1
  In1/1 -> Selector/1
  Compare To Constant/1 -> Assertion/1
